simulink model "Drone_simulation_PX4"  (R2025b)
settings: Solver=FixedStepAuto  StartTime=0.0  StopTime=inf  RelTol=1e-6
undefined symbols (not defined in the file): CommParams, fractalcoef, g, Gravity, HIL_GPS_Ts, HIL_HEARTBEAT_Ts, HIL_SENSOR_Ts, HIL_STATE_QUATERNION_Ts, IC, omega_max, Payload, PhysicalScaling, rho_0, SimParams, tau_motor, Tmax_total, Total_mass
libraries: uavmavlinklib x25, slrealtimeiplib x6, sim3dlib x4, aerolibatmos2 x2, matrix_library x1, simulink_extras x1, aerolibasang x1, sensorgpslib x1, mspsensorlib x1, sharedutil x1, aerolibconvert2 x1
(part 3 of 3)

== matlab function Drone_simulation_PX4/Drone Model/Matchematical Drone Model/MATLAB Function3 ==
  data: is_new input; m_out output; m_px4 input; u_hover_cmd input; ready output
function [m_out, ready] = px4_motor_interface(is_new, m_px4, u_hover_cmd)
%#codegen
%
% PX4 motor-command interface.
%
% - Detects when PX4 begins producing meaningful motor commands
% - Requires several consecutive valid packets before takeover
% - Latches PX4 takeover
% - Holds the latest valid PX4 motor command between packets
% - Smoothly transitions from initial hover command to PX4
%
% Inputs:
%   is_new       New MAVLink actuator packet flag
%   m_px4        PX4 motor commands [4 elements]
%   u_hover_cmd  Stable initial hover commands [4 elements]
%
% Outputs:
%   m_out        Motor commands to plant [4x1]
%   ready        1 once PX4 takeover has occurred

persistent ready_latched
persistent m_hold
persistent alpha
persistent ready_count

%% Parameters

Ts          = single(0.0001);
ramp_time   = single(2.0);

% PX4 must command at least this fraction of hover collective
% before takeover is allowed.
ready_fraction = single(0.5);

% Number of consecutive valid/meaningful packets required
required_packets = uint16(10);

%% Input formatting

m_px4 = reshape(single(m_px4), 4, 1);

u_hover_cmd = reshape( ...
    single(u_hover_cmd), 4, 1);

new_packet = is_new ~= 0;

%% Initialize persistent states

if isempty(ready_latched)
    ready_latched = false;
end

if isempty(m_hold)
    m_hold = u_hover_cmd;
end

if isempty(alpha)
    alpha = single(0);
end

if isempty(ready_count)
    ready_count = uint16(0);
end

%% Validate received PX4 command

packet_valid = ...
    new_packet && ...
    all(isfinite(m_px4)) && ...
    all(m_px4 >= single(0)) && ...
    all(m_px4 <= single(1));

%% Determine whether PX4 is producing meaningful collective thrust

hover_level = mean(u_hover_cmd);
px4_level   = mean(m_px4);

collective_ready = ...
    px4_level >= ready_fraction * hover_level;

%% Require several consecutive meaningful packets

if ~ready_latched

    if packet_valid && collective_ready

        if ready_count < required_packets
            ready_count = ready_count + uint16(1);
        end

    else
        ready_count = uint16(0);
    end

    %% Latch takeover

    if ready_count >= required_packets
        ready_latched = true;

        % Start blending from current hover command
        alpha = single(0);

        % Store current valid PX4 command
        m_hold = m_px4;
    end
end

%% Before PX4 takeover

if ~ready_latched

    m_hold = u_hover_cmd;
    alpha  = single(0);

    m_out = u_hover_cmd;
    ready = false;

    return;
end

%% Hold most recently received valid PX4 command

if packet_valid
    m_hold = m_px4;
end

%% Smooth transition from hover to PX4

alpha = min( ...
    alpha + Ts/ramp_time, ...
    single(1));

m_out = ...
    (single(1) - alpha).*u_hover_cmd + ...
    alpha.*m_hold;

%% Safety saturation

m_out = min( ...
    max(m_out, single(0)), ...
    single(1));

ready = true;

end

== matlab function Drone_simulation_PX4/Drone Model/Matchematical Drone Model/Drone Dynamics/Mechnical System/Translational Mechanics /Ground Force ==
  data: S input; F_ground output; S_dot input
function F_ground = ground_contact(S, S_dot)
%#codegen

z     = S(3);
z_dot = S_dot(3);

k_ground = 2000.0;  % [N/m]
c_ground = 100.0;   % [N/(m/s)]

penetration = -z;

if penetration > 0
    Fz = k_ground*penetration - c_ground*z_dot;

    % Ground can push up, but not pull down
    if Fz < 0
        Fz = 0;
    end
else
    Fz = 0;
end

F_ground = [0; 0; Fz];
end

== matlab function Drone_simulation_PX4/Drone Model/Matchematical Drone Model/ENU to NED/MATLAB Function ==
  data: S_enu input; S_ned output; Sdot_enu input; Sddot_enu input; Omega_flu input; Eta_enu input; R_enu input; Sdot_ned output; Sddot_ned output; Omega_frd output; Omega_nav_ned output; Eta_ned output; R_ned output; R_ned_to_frd output
function [S_ned, Sdot_ned, Sddot_ned, ...
          Omega_frd, Omega_nav_ned, ...
          Eta_ned, R_ned, R_ned_to_frd] = ...
    enu2ned_full(S_enu, Sdot_enu, Sddot_enu, ...
                 Omega_flu, Eta_enu, R_enu)

%#codegen

%% ------------------------------------------------------------------------
% Force input dimensions
% -------------------------------------------------------------------------

S_enu     = reshape(S_enu,     [3 1]);
Sdot_enu  = reshape(Sdot_enu,  [3 1]);
Sddot_enu = reshape(Sddot_enu, [3 1]);

Omega_flu = reshape(Omega_flu, [3 1]);
Eta_enu   = reshape(Eta_enu,   [3 1]);

R_enu = reshape(R_enu, [3 3]);


%% ------------------------------------------------------------------------
% Explicitly define output sizes
% -------------------------------------------------------------------------

S_ned         = zeros(3,1);
Sdot_ned      = zeros(3,1);
Sddot_ned     = zeros(3,1);

Omega_frd     = zeros(3,1);
Omega_nav_ned = zeros(3,1);

Eta_ned       = zeros(3,1);

R_ned         = zeros(3,3);
R_ned_to_frd  = zeros(3,3);


%% ------------------------------------------------------------------------
% ENU navigation frame -> NED navigation frame
% -------------------------------------------------------------------------

T = [ ...
     0  1  0;
     1  0  0;
     0  0 -1];


%% ------------------------------------------------------------------------
% FLU body frame -> FRD body frame
% -------------------------------------------------------------------------

B = [ ...
     1  0  0;
     0 -1  0;
     0  0 -1];


%% ------------------------------------------------------------------------
% Translational quantities
% -------------------------------------------------------------------------

S_ned = ...
    T * S_enu;

Sdot_ned = ...
    T * Sdot_enu;

Sddot_ned = ...
    T * Sddot_enu;


%% ------------------------------------------------------------------------
% Body angular velocity
% -------------------------------------------------------------------------

Omega_frd = ...
    B * Omega_flu;


%% ------------------------------------------------------------------------
% Rotation matrices
% -------------------------------------------------------------------------

% FRD body -> NED navigation frame
R_ned = ...
    T * R_enu * B;

% NED navigation frame -> FRD body frame
R_ned_to_frd = ...
    R_ned.';


%% ------------------------------------------------------------------------
% Angular velocity expressed in NED navigation frame
% -------------------------------------------------------------------------

Omega_nav_ned = ...
    R_ned * Omega_frd;


%% ------------------------------------------------------------------------
% Extract NED Euler angles
%
% ZYX convention:
%
%   psi   = yaw
%   theta = pitch
%   phi   = roll
%
% Output order is deliberately:
%
%   Eta_ned = [yaw; pitch; roll]
%
% so it can be fed directly into a ZYX
% Rotation Angles to Quaternions block.
% -------------------------------------------------------------------------

theta_ned = ...
    asin_sat(-R_ned(3,1));

phi_ned = ...
    atan2( ...
        R_ned(3,2), ...
        R_ned(3,3));

psi_ned = ...
    atan2( ...
        R_ned(2,1), ...
        R_ned(1,1));

Eta_ned = [ ...
    psi_ned;
    theta_ned;
    phi_ned];


%% ------------------------------------------------------------------------
% Enforce final dimensions
% -------------------------------------------------------------------------

S_ned         = reshape(S_ned,         [3 1]);
Sdot_ned      = reshape(Sdot_ned,      [3 1]);
Sddot_ned     = reshape(Sddot_ned,     [3 1]);

Omega_frd     = reshape(Omega_frd,     [3 1]);
Omega_nav_ned = reshape(Omega_nav_ned, [3 1]);

Eta_ned       = reshape(Eta_ned,       [3 1]);

R_ned         = reshape(R_ned,         [3 3]);
R_ned_to_frd  = reshape(R_ned_to_frd,  [3 3]);

% Eta_enu is intentionally unused at the moment.

end


function y = asin_sat(x)

x = min(max(x, -1), 1);

y = asin(x);

end

== matlab function Drone_simulation_PX4/Drone Model/Matchematical Drone Model/Drone Dynamics/Mechnical System/Rotational Mechanics/Euler Rate Matrix ==
  data: roll input; Tmat output; pitch input
function Tmat = eulerRateMatrix(roll, pitch)
phi   = roll;
theta = pitch;

Tmat = [ ...
    1,  sin(phi)*tan(theta),        cos(phi)*tan(theta);
    0,  cos(phi),                  -sin(phi);
    0,  sin(phi)/cos(theta),        cos(phi)/cos(theta) ];
end

== matlab function Drone_simulation_PX4/Drone Model/Matchematical Drone Model/Drone Dynamics/Mechnical System/Translational Mechanics /Rotation Matric ==
  data: roll input; R_IB output; pitch input; yaw input
function R_IB = rotmat(roll, pitch, yaw)
phi   = roll;
theta = pitch;
psi   = yaw;

R_IB = [ ...
    cos(psi)*cos(theta),  cos(psi)*sin(theta)*sin(phi) - sin(psi)*cos(phi),  cos(psi)*sin(theta)*cos(phi) + sin(psi)*sin(phi);
    sin(psi)*cos(theta),  sin(psi)*sin(theta)*sin(phi) + cos(psi)*cos(phi),  sin(psi)*sin(theta)*cos(phi) - cos(psi)*sin(phi);
   -sin(theta),           cos(theta)*sin(phi),                               cos(theta)*cos(phi) ];
end

== matlab function Drone_simulation_PX4/From PX4/MATLAB Function ==
  settings: updateMethod=DISCRETE
  data: isNew input; ready_out output; motors input; tau_x input; tau_y input; tau_z input; T_mix input
function ready_out = px4_ready_latch( ...
    isNew, motors, tau_x, tau_y, tau_z, T_mix)
%#codegen

persistent ready good_packets

if isempty(ready)
    ready = false;
    good_packets = uint16(0);
end

% Extract the four PX4 motor commands
m1 = single(motors(1));
m2 = single(motors(2));
m3 = single(motors(3));
m4 = single(motors(4));

is_new = isNew ~= 0;

%% Check the received motor command

motors_finite = ...
    isfinite(m1) && isfinite(m2) && ...
    isfinite(m3) && isfinite(m4);

motors_in_range = ...
    m1 >= single(0) && m1 <= single(1) && ...
    m2 >= single(0) && m2 <= single(1) && ...
    m3 >= single(0) && m3 <= single(1) && ...
    m4 >= single(0) && m4 <= single(1);

motor_mean = single(0.25) * (m1 + m2 + m3 + m4);

motor_max = max(max(m1,m2), max(m3,m4));
motor_min = min(min(m1,m2), min(m3,m4));

motor_spread = motor_max - motor_min;

%% Check the converted plant inputs

outputs_finite = ...
    isfinite(T_mix) && ...
    isfinite(tau_x) && ...
    isfinite(tau_y) && ...
    isfinite(tau_z);

T_hover = single(15.0);

% PX4 must actually be producing thrust
motors_active = ...
    motor_mean > single(0.08) && ...
    motor_mean < single(0.75);

% Broad thrust limits; these are only sanity checks
thrust_sane = ...
    T_mix > single(0.30)*T_hover && ...
    T_mix < single(2.00)*T_hover;

% Avoid handing over while PX4 is completely saturated
distribution_sane = motor_spread < single(0.40);

packet_valid = ...
    is_new && ...
    motors_finite && ...
    motors_in_range && ...
    outputs_finite && ...
    motors_active && ...
    thrust_sane && ...
    distribution_sane;

%% Require several valid MAVLink packets

if ~ready

    if packet_valid
        if good_packets < uint16(1000)
            good_packets = good_packets + uint16(1);
        end
    else
        good_packets = uint16(0);
    end

    % 20 valid new packets before takeover
    if good_packets >= uint16(20)
        ready = true;
    end
end

ready_out = double(ready);

end

== matlab function Drone_simulation_PX4/Debugger/MATLAB Function ==
  data: S output; S_dot output; S_ddot output; Omega output; Eta output; Orientation output
function [S, S_dot, S_ddot, Omega, Eta, Orientation] = fixed_hover_state()
%#codegen
% Fixed ideal hover state for debugging PX4 sensor input.
%
% ENU world:
%   x = East
%   y = North
%   z = Up
%
% Body assumed FLU:
%   x = Forward
%   y = Left
%   z = Up

% Position [m]
S = [0; 0; 1];

% Velocity [m/s]
S_dot = [0; 0; 0];

% Translational acceleration [m/s^2]
% Keep zero for the state. IMU specific force is handled separately.
S_ddot = [0; 0; 0];

% Euler angles [roll; pitch; yaw] [rad]
% yaw = pi/2 gives PX4/NED yaw ≈ 0 after ENU->NED conversion.
Eta = [0; 0; pi/2];

% Body angular rates [p; q; r] [rad/s]
Omega = [0; 0; 0];

% Body-to-world ENU rotation matrix
roll  = Eta(1);
pitch = Eta(2);
yaw   = Eta(3);

Orientation = rotmat(roll, pitch, yaw);

end


function R_IB = rotmat(roll, pitch, yaw)
phi   = roll;
theta = pitch;
psi   = yaw;

R_IB = [ ...
    cos(psi)*cos(theta),  cos(psi)*sin(theta)*sin(phi) - sin(psi)*cos(phi),  cos(psi)*sin(theta)*cos(phi) + sin(psi)*sin(phi);
    sin(psi)*cos(theta),  sin(psi)*sin(theta)*sin(phi) + cos(psi)*cos(phi),  sin(psi)*sin(theta)*cos(phi) - cos(psi)*sin(phi);
   -sin(theta),           cos(theta)*sin(phi),                               cos(theta)*cos(phi) ];
end

== matlab function Drone_simulation_PX4/Debugger/TCP // MAVLink Send Subsystem1/HIL STATE QUATERNION/MATLAB Function ==
  data: attitude_quaternion output; rollspeed output; pitchspeed output; yawspeed output; lat output; lon output; alt output; vx output; vy output; vz output; ind_airspeed output; true_airspeed output; xacc output; yacc output; zacc output
function [attitude_quaternion, ...
          rollspeed, pitchspeed, yawspeed, ...
          lat, lon, alt, ...
          vx, vy, vz, ...
          ind_airspeed, true_airspeed, ...
          xacc, yacc, zacc] = fixed_hil_state_quaternion()
%#codegen
% Fixed HIL_STATE_QUATERNION for PX4 diagnostic.
%
% MAVLink HIL_STATE_QUATERNION units:
% attitude_quaternion: [w x y z], size [1x4]
% rollspeed/pitchspeed/yawspeed: [rad/s]
% lat/lon: degrees * 1e7
% alt: millimeters above mean sea level
% vx/vy/vz: velocity [cm/s] in NED
% ind_airspeed/true_airspeed: [cm/s]
% xacc/yacc/zacc: acceleration [mG]

% ---------------------------------------------------------
% Attitude
% ---------------------------------------------------------

% Level attitude in PX4 NED/FRD convention.
% IMPORTANT: this must be a ROW vector [1x4], not [4x1].
attitude_quaternion = single([1 0 0 0]);

% Body angular rates [rad/s]
rollspeed  = single(0.0);
pitchspeed = single(0.0);
yawspeed   = single(0.0);

% ---------------------------------------------------------
% Position
% ---------------------------------------------------------

lat0_deg = 55.785;
lon0_deg = 12.521;
alt_m = 51.0;

lat = int32(lat0_deg * 1e7);
lon = int32(lon0_deg * 1e7);
alt = int32(alt_m * 1000);     % [mm] AMSL

% ---------------------------------------------------------
% Velocity in NED [cm/s]
% ---------------------------------------------------------

vx = int16(0);
vy = int16(0);
vz = int16(0);

% ---------------------------------------------------------
% Airspeed [cm/s]
% ---------------------------------------------------------

ind_airspeed  = uint16(0);
true_airspeed = uint16(0);

% ---------------------------------------------------------
% Acceleration [mG]
% ---------------------------------------------------------

xacc = int16(0);
yacc = int16(0);
zacc = int16(-1000);

end
